simulink model "vRTHS_2024"  (R2025b)
settings: Solver=ode4  StartTime=0.0  StopTime=tend  FixedStep=dt_rths  RelTol=1e-3  EnableMultiTasking=on
values from neighbouring files (symbols this model uses):
  a1_beta0 = 2.1283e+13    (= 21283000000000)    [F1_input_file.m]
  a2 = 4.2297e+06    (= 4229700)    [F1_input_file.m]
  a3 = 3.3        + 1.3   * nom *randn(1,1)    [F1_input_file.m]
  A_ns = [     zeros(n) eye(n) ... (first row only)    [F1_input_file.m]
  AA_R = [zeros(dof)        eye(dof) ... (first row only)    [F1_Modifications.m]
  B_ns = [     zeros(n,1)      zeros(n) ... (first row only)    [F1_input_file.m]
  b_th = 0.13    [RUN_vRTHS_demo_new.m]
  BB_R = [zeros(dof,1) ... (first row only)    [F1_Modifications.m]
  beta1 = 425        + 3.3   * nom *randn(1,1)    [F1_input_file.m]
  beta2 = 9.9976e+04 + 3.3e3 * nom *randn(1,1)    [F1_input_file.m]
  c_e = 2*z_e*m_e*sqrt(KE(1,1)/m_e)    [F1_input_file.m]
  C_ns = [     eye(n)              zeros(n) ... (first row only)    [F1_input_file.m]
  CC_R = [ eye(dof)   zeros(dof) ... (first row only)    [F1_Modifications.m]
  CE = zeros(n)    [F1_input_file.m]
  consider_damage = 0    [RUN_vRTHS_demo_new.m]
  D_ns = [     zeros(n,1)            zeros(n) ... (first row only)    [F1_input_file.m]
  DD_R = [zeros(2*dof,1) ... (first row only)    [F1_Modifications.m]
  dt_rths = 0.000244140625    [Plant.mat]    (also in RUN_vRTHS_demo_new.m)
  E_sw = 1    [F1_input_file.m]
  eq_intensity = .4    (= 0.4)    [F1_input_file.m]
  fs = 4096    [RUN_vRTHS_demo_new.m]
  gain = 1.0261    [F1_input_file.m]
  Gsnsr_DT = 1    [F1_input_file.m]
  Gsnsr_FT = 1    [F1_input_file.m]
  k_e = 1190e3    (= 1190000)    [F1_input_file.m]
  KE = zeros(n)    [F1_input_file.m]
  m_e = m_e*1.3    [F1_Modifications.m]    (also in F1_input_file.m = 29.13)
  ME = ME*1.3    [F1_Modifications.m]    (also in F1_input_file.m = zeros(n))
  modified = 1    [RUN_vRTHS_demo_new.m]
  sat_limit_lower = -3.8    [F1_input_file.m]
  sat_limit_upper = +3.8    (= 3.8)    [F1_input_file.m]
  Seed_snr = rng(seed)    [F1_input_file.m]
  tend = 90    [F1_input_file.m]
undefined symbols (not defined in the file or in its folder): Acd, Apred_mod, Bcd, Bpred_mod, Ccd, Cpred_mod, Dcd, digital_cntrlr, digital_cntrlr2, Dpred_mod
libraries: simulink x3, cstblocks x1, rtwinlib x1
settings Model: SimulationMode=accelerator  Creator=IISL_0175  LastModifiedBy=Victus
settings SolverCC: AlgebraicLoopSolver=TrustRegion
settings DataIOCC: SaveFormat=StructureWithTime  ReturnWorkspaceOutputs=off
settings OptimizationCC: LifeSpan=inf
settings DebuggingCC: InheritedTsInSrcMsg=none  UnconnectedInputMsg=warning  UnconnectedOutputMsg=warning  UnconnectedLineMsg=warning  SFUnexpectedBacktrackingDiag=warning  SFNoUnconditionalDefaultTransitionDiag=warning  SFExecutionAtInitializationDiag=none  ArithmeticOperatorsInVariantConditions=warning
settings HardwareCC: ProdBitPerSizeT=32.0  ProdBitPerPtrDiffT=32.0  ProdWordSize=32.0  ProdHWDeviceType=Specified
settings SFSimCC: SimUseLocalCustomCode=off  CustomCodeUndefinedFunction=UseInterfaceOnly
settings RTWCC: RTWUseLocalCustomCode=off  GPUComputeCapability=3.5
settings CodeAppCC: StateflowObjectComments=on
settings GRTTargetCC: TargetLangStandard=C89/C90 (ANSI)
settings ConfigComp: CovMetricSettings=dw  CovSaveCumulativeToWorkspaceVar=on  CovSaveSingleToWorkspaceVar=on  CovExternalEMLEnable=off

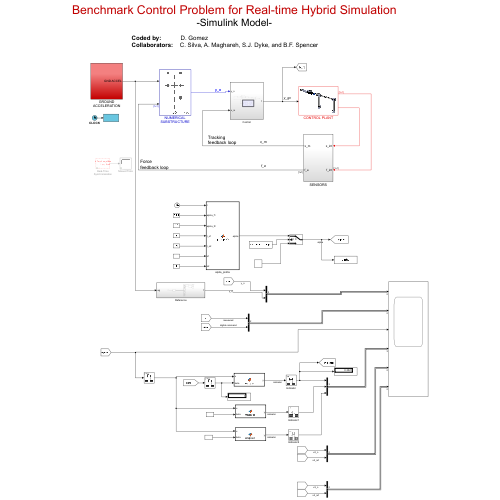
[thumbnail: Simulink's stored preview of the top-level diagram]
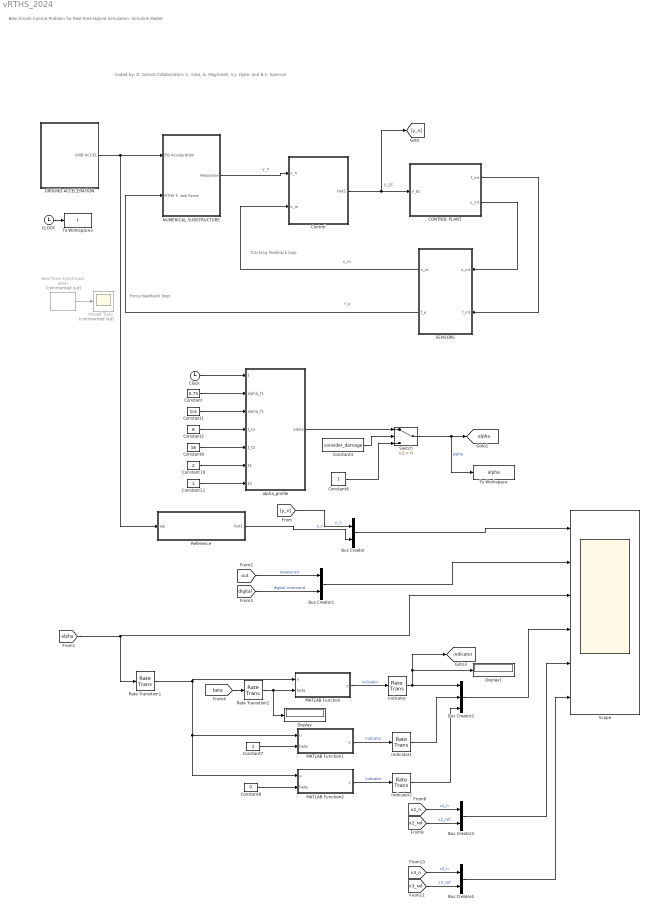
== system vRTHS_2024 ==
  note: Force
      | feedback loop
  note: Benchmark Control Problem for Real-time Hybrid Simulation
      | -Simulink Model-
  note: Coded by: D. Gomez
      | Collaborators: C. Silva, A. Maghareh, S.J. Dyke, and B.F. Spencer
  note: Tracking feedback loop
  note: y_n
  note: y_gc
  note: f_e
  note: x_m
  Bus Creator{,1,3..4} (4 alike) : BusCreator  Inputs=2
  Bus Creator2 : BusCreator  Inputs=3
  CLOCK : Clock
  CONTROL PLANT : Subsystem
      mask Display: image(imread('PlantSW2.PNG'));
  Clock : Clock
  Constant : Constant  Value=0.75
  Constant1 : Constant  Value=0.5
  Constant10 : Constant  Value=2
  Constant11 : Constant
  Constant2 : Constant  Value=8
  Constant3 : Constant  Value=consider_damage
  Constant6 : Constant
  Constant7 : Constant
  Constant8 : Constant  Value=0
  Constant9 : Constant  Value=16
  Control : Subsystem
  Display : Display
  Display1 : Display
  GROUND ACCELERATION : Subsystem
  Indicator : RateTransition
  Indicator1 : RateTransition
  Indicator2 : RateTransition
  MATLAB Function : MATLAB Function  TreatAsAtomicUnit=on  SystemSampleTime=100/fs
  MATLAB Function1 : MATLAB Function  TreatAsAtomicUnit=on  SystemSampleTime=100/fs
  MATLAB Function2 : MATLAB Function  TreatAsAtomicUnit=on  SystemSampleTime=100/fs
  Missed Ticks : Scope  Commented=on
      settings: TimeSpan=10  ActiveDisplayYMinimum=-51.75  ActiveDisplayYMaximum=465.75  DataLoggingSaveFormat=Structure
  NUMERICAL SUBSTRUCTURE : Subsystem
      mask Display: image(imread('Num_sub.png'));
  Rate Transition1 : RateTransition
  Rate Transition2 : RateTransition
  Real-Time Synchronization : rtwinlib/Real-Time Synchronization  Commented=on  SampleTime=dt_rths  MaxMissedTicks=10000  ShowMissedTicks=on  YieldWhenWaiting=off
  Reference : Subsystem
  SENSORS : Subsystem
  Scope : Scope  NumInputPorts=6
      settings: ActiveDisplayString=3  ActiveDisplayYMinimum=0.9  ActiveDisplayYMaximum=1.1  DataLoggingVariableName=ScopeData5
  Switch : Switch  Criteria=u2 > Threshold  SaturateOnIntegerOverflow=off  InputSameDT=off
  To Workspace : ToWorkspace  VariableName=alpha  SaveFormat=Timeseries  SampleTime=-1
  To Workspace3 : ToWorkspace  VariableName=t  SampleTime=-1
  alpha_profile : MATLAB Function  TreatAsAtomicUnit=on
  tag scope: alpha=global, indicator=global
  wires:
  CLOCK/1 -> To Workspace3/1
  CONTROL PLANT/2(x_int) -> SENSORS/1(x_int)
  SENSORS/2("f_e ") -> NUMERICAL SUBSTRUCTURE/2(RTHS feedback Force)
  Control/1(Out1) -> [y_n], CONTROL PLANT/1(y_gc)
  Real-Time Synchronization/1 -> Missed Ticks/1
  GROUND ACCELERATION/1(GND ACCEL) -> Reference/1(ag), NUMERICAL SUBSTRUCTURE/1(EQ Acceleration)
  CONTROL PLANT/1(f_int) -> SENSORS/2(f_int)
  Switch/1 -> To Workspace/1, [alpha]  "alpha"
  Constant/1 -> alpha_profile/2(alpha_f1)
  Clock/1 -> alpha_profile/1(t)
  alpha_profile/1(alpha) -> Switch/1
  Constant11/1 -> alpha_profile/7(k2)
  Constant1/1 -> alpha_profile/3(alpha_f2)
  Constant6/1 -> Switch/3
  Constant2/1 -> alpha_profile/4(t_s1)
  Constant9/1 -> alpha_profile/5(t_s2)
  Constant10/1 -> alpha_profile/6(k1)
  Bus Creator3/1 -> Scope/5
  Bus Creator2/1 -> Scope/4
  MATLAB Function/1(y) -> Indicator/1  "indicator"
  Indicator1/1 -> Bus Creator2/2
  Bus Creator1/1 -> Scope/2
  Bus Creator4/1 -> Scope/6
  Rate Transition1/1 -> MATLAB Function2/1(u), MATLAB Function1/1(u), MATLAB Function/1(u)
  Bus Creator/1 -> Scope/1
  Rate Transition2/1 -> Display/1, MATLAB Function/2(beta)
  Constant7/1 -> MATLAB Function1/2(beta)
  [digital] -> Bus Creator1/2  "digital command"
  [x3_n] -> Bus Creator4/1  "x3_n"
  [x3_ref] -> Bus Creator4/2  "x3_ref"
  [x2_ref] -> Bus Creator3/2  "x2_ref"
  [out] -> Bus Creator1/1  "measured"
  [y_n] -> Bus Creator/1  "y_n"
  Constant8/1 -> MATLAB Function2/2(beta)
  [x2_n] -> Bus Creator3/1  "x2_n"
  [alpha] -> Rate Transition1/1, Scope/3
  MATLAB Function1/1(y) -> Indicator1/1  "indicator"
  Indicator2/1 -> Bus Creator2/3
  Reference/1(Out1) -> Bus Creator/2  "y_r"
  Indicator/1 -> [indicator], Display1/1, Bus Creator2/1
  [beta] -> Rate Transition2/1
  MATLAB Function2/1(y) -> Indicator2/1  "indicator"
  SENSORS/1(x_m) -> Control/2(x_m)
  NUMERICAL SUBSTRUCTURE/1(Response) -> Control/1(y_n)
  Constant3/1 -> Switch/2

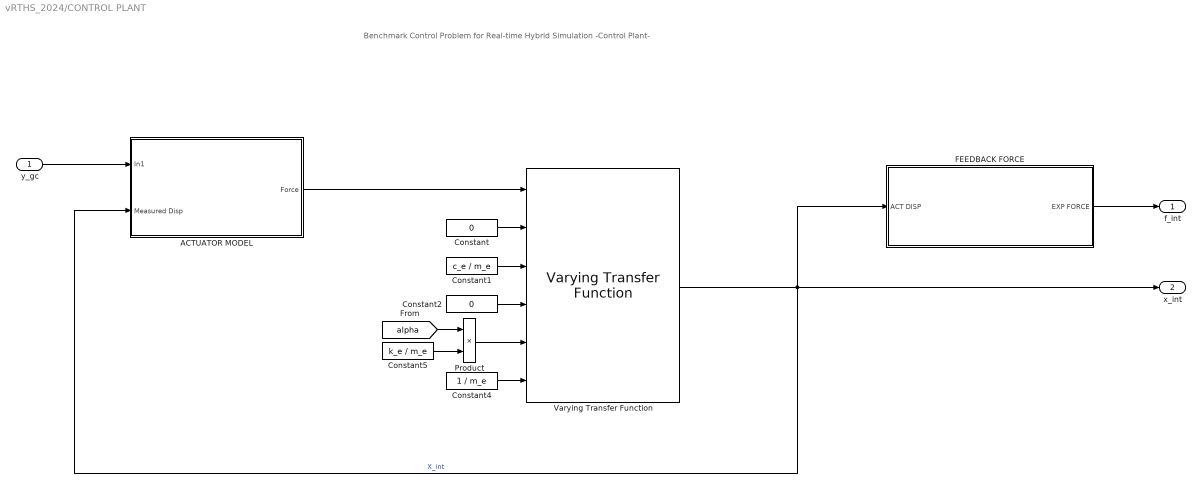
== system vRTHS_2024/CONTROL PLANT ==
  note: Benchmark Control Problem for Real-time Hybrid Simulation
      | -Control Plant-
  y_gc : Inport
  ACTUATOR MODEL : Subsystem
      mask Display: image(imread('ActuatorSW2.PNG'));
  Constant : Constant  Value=0
  Constant1 : Constant  Value=c_e / m_e
  Constant2 : Constant  Value=0
  Constant4 : Constant  Value=1 / m_e
  Constant5 : Constant  Value=k_e / m_e
  FEEDBACK FORCE : Subsystem
  Product : Product
  Varying Transfer Function : cstblocks/Linear Parameter Varying/Varying Transfer Function  N=2  Feedthrough=on
  f_int : Outport
  x_int : Outport  Port=2
  wires:
  y_gc/1 -> ACTUATOR MODEL/1(In1)
  Varying Transfer Function/1 -> FEEDBACK FORCE/1(ACT DISP), x_int/1, ACTUATOR MODEL/2(Measured Disp)  "X_int"
  ACTUATOR MODEL/1(Force) -> Varying Transfer Function/1
  FEEDBACK FORCE/1(EXP FORCE) -> f_int/1
  Constant4/1 -> Varying Transfer Function/6
  [alpha] -> Product/1
  Product/1 -> Varying Transfer Function/5
  Constant1/1 -> Varying Transfer Function/3
  Constant5/1 -> Product/2
  Constant/1 -> Varying Transfer Function/2
  Constant2/1 -> Varying Transfer Function/4

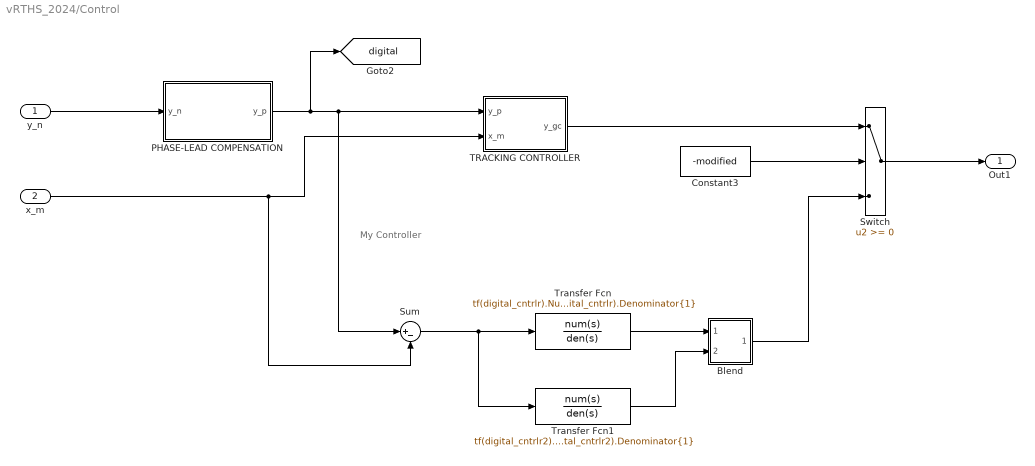
== system vRTHS_2024/Control ==
  note: My Controller
  y_n : Inport
  x_m : Inport  Port=2
  Blend : Subsystem
  Constant3 : Constant  Value=-modified
  PHASE-LEAD COMPENSATION : Subsystem
  Sum : Sum  Inputs=|+-
  Switch : Switch  SaturateOnIntegerOverflow=off  InputSameDT=off
  TRACKING CONTROLLER : Subsystem
  Transfer Fcn : TransferFcn  Numerator=tf(digital_cntrlr).Numerator{1}  Denominator=tf(digital_cntrlr).Denominator{1}
  Transfer Fcn1 : TransferFcn  Numerator=tf(digital_cntrlr2).Numerator{1}  Denominator=tf(digital_cntrlr2).Denominator{1}
  Out1 : Outport
  tag scope: digital=global
  wires:
  x_m/1 -> Sum/2, TRACKING CONTROLLER/2(x_m)
  Sum/1 -> Transfer Fcn1/1, Transfer Fcn/1
  Transfer Fcn1/1 -> Blend/2(In2)
  Transfer Fcn/1 -> Blend/1(In1)
  TRACKING CONTROLLER/1(y_gc) -> Switch/1
  Blend/1(Out1) -> Switch/3
  PHASE-LEAD COMPENSATION/1(y_p) -> [digital], Sum/1, TRACKING CONTROLLER/1(y_p)
  Constant3/1 -> Switch/2
  Switch/1 -> Out1/1
  y_n/1 -> PHASE-LEAD COMPENSATION/1(y_n)

== system vRTHS_2024/GROUND ACCELERATION ==
  note: Benchmark Control Problem for Real-time Hybrid Simulation
      | -Ground Acceleration-
  GROUND ACCELERATION : ToWorkspace  VariableName=EQ_input  SampleTime=-1
  INPUT SELECTOR : MultiPortSwitch  Inputs=4  SaturateOnIntegerOverflow=off  InputSameDT=off
  "RECORD " : Subsystem
  SCALING : Gain  Gain=eq_intensity  Multiplication=Matrix(K*u)
  SWITCH CONSTANT : Constant  Value=E_sw
  GND ACCEL : Outport
  wires:
  INPUT SELECTOR/1 -> SCALING/1
  SWITCH CONSTANT/1 -> INPUT SELECTOR/1
  "RECORD "/1(El Centro) -> INPUT SELECTOR/2
  "RECORD "/2(Kobe) -> INPUT SELECTOR/3
  "RECORD "/3(Morgan) -> INPUT SELECTOR/4
  SCALING/1 -> GROUND ACCELERATION/1, GND ACCEL/1
  "RECORD "/4(Chirp) -> INPUT SELECTOR/5

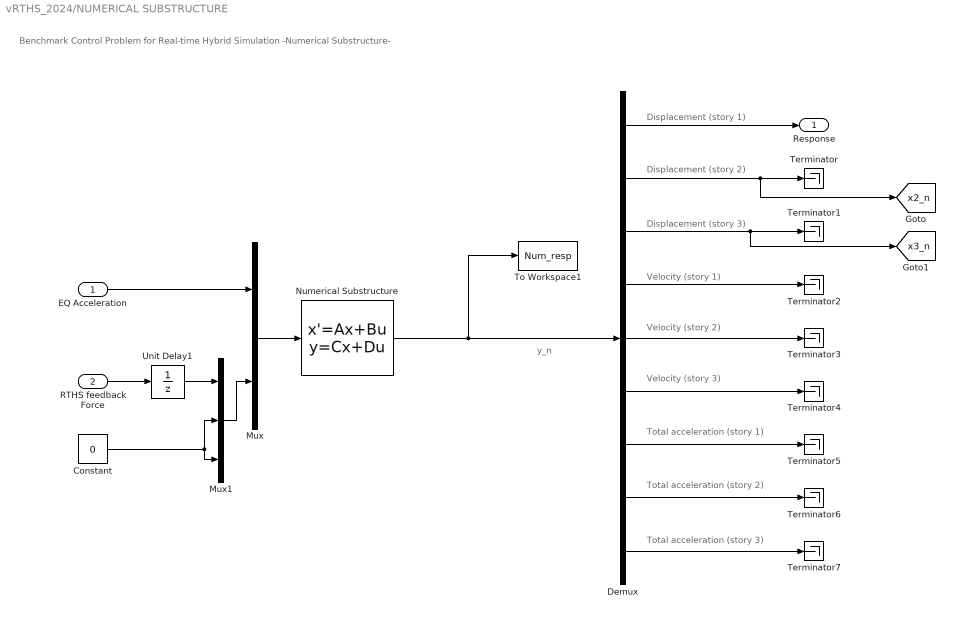
== system vRTHS_2024/NUMERICAL SUBSTRUCTURE ==
  note: y_n
  note: Benchmark Control Problem for Real-time Hybrid Simulation
      | -Numerical Substructure-
  note: Velocity (story 3)
  note: Displacement (story 3)
  note: Displacement (story 1)
  note: Total acceleration (story 1)
  note: Velocity (story 1)
  note: Velocity (story 2)
  note: Total acceleration (story 3)
  note: Displacement (story 2)
  note: Total acceleration (story 2)
  EQ Acceleration : Inport
  RTHS feedback Force : Inport  Port=2
  Constant : Constant  Value=0
  Demux : Demux  Outputs=9
  Mux : Mux  Inputs=2
  Mux1 : Mux  Inputs=3
  Numerical Substructure : StateSpace  A=A_ns  B=B_ns  C=C_ns  D=D_ns  InitialCondition=0
  Terminator{,1..7} (8 alike) : Terminator
  To Workspace1 : ToWorkspace  VariableName=Num_resp  SaveFormat=Timeseries  SampleTime=-1
  Unit Delay1 : UnitDelay  SampleTime=-1  HasFrameUpgradeWarning=on
  Response : Outport
  tag scope: x2_n=global, x3_n=global
  wires:
  Mux/1 -> Numerical Substructure/1
  EQ Acceleration/1 -> Mux/1
  RTHS feedback Force/1 -> Unit Delay1/1
  Numerical Substructure/1 -> To Workspace1/1, Demux/1
  Demux/2 -> [x2_n], Terminator/1
  Demux/7 -> Terminator5/1
  Demux/8 -> Terminator6/1
  Demux/9 -> Terminator7/1
  Demux/4 -> Terminator2/1
  Demux/6 -> Terminator4/1
  Demux/5 -> Terminator3/1
  Demux/1 -> Response/1
  Demux/3 -> [x3_n], Terminator1/1
  Constant/1 -> Mux1/2, Mux1/3
  Mux1/1 -> Mux/2
  Unit Delay1/1 -> Mux1/1

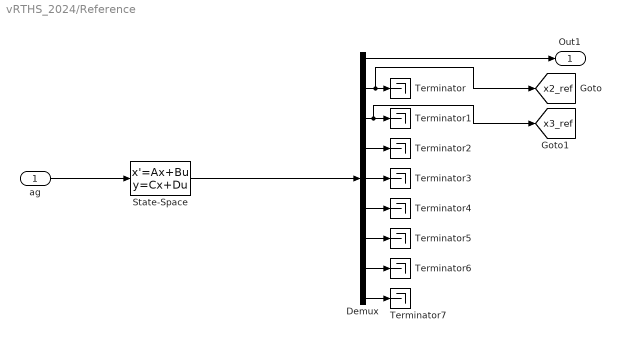
== system vRTHS_2024/Reference ==
  ag : Inport
  Demux : Demux  Outputs=9
  State-Space : StateSpace  A=AA_R  B=BB_R  C=CC_R  D=DD_R  InitialCondition=0
  Terminator{,1..7} (8 alike) : Terminator
  Out1 : Outport
  tag scope: x2_ref=global, x3_ref=global
  wires:
  Demux/7 -> Terminator5/1
  Demux/6 -> Terminator4/1
  Demux/8 -> Terminator6/1
  Demux/9 -> Terminator7/1
  Demux/3 -> [x3_ref], Terminator1/1
  Demux/4 -> Terminator2/1
  Demux/2 -> [x2_ref], Terminator/1
  Demux/5 -> Terminator3/1
  State-Space/1 -> Demux/1
  ag/1 -> State-Space/1
  Demux/1 -> Out1/1

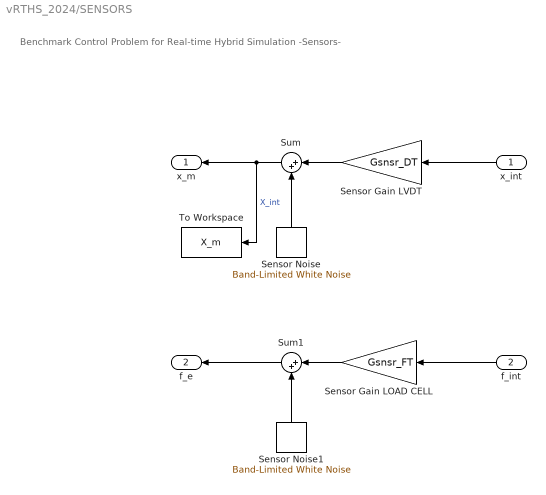
== system vRTHS_2024/SENSORS ==
  note: Benchmark Control Problem for Real-time Hybrid Simulation
      | -Sensors-
  x_int : Inport
  f_int : Inport  Port=2
  Sensor Noise : simulink/Sources/Band-Limited White Noise  Cov=rms_noise_DT  Ts=dt_rths  seed=double(Seed_snr.Seed)
  Sensor Noise1 : simulink/Sources/Band-Limited White Noise  Cov=rms_noise_FT  Ts=dt_rths  seed=double(Seed_snr.Seed)
  Sensor Gain LVDT : Gain  Gain=Gsnsr_DT  SaturateOnIntegerOverflow=on  OutDataTypeStr=Inherit: Same as input  ParamDataTypeStr=Inherit: Same as input
  Sensor Gain LOAD CELL : Gain  Gain=Gsnsr_FT  SaturateOnIntegerOverflow=on  OutDataTypeStr=Inherit: Same as input  ParamDataTypeStr=Inherit: Same as input
  Sum : Sum  Inputs=|++  InputSameDT=on  SaturateOnIntegerOverflow=on  OutDataTypeStr=Inherit: Same as first input
  Sum1 : Sum  Inputs=|++  InputSameDT=on  SaturateOnIntegerOverflow=on  OutDataTypeStr=Inherit: Same as first input
  To Workspace : ToWorkspace  VariableName=X_m  SaveFormat=Timeseries  SampleTime=-1
  x_m : Outport
  "f_e " : Outport  Port=2
  wires:
  Sensor Gain LVDT/1 -> Sum/1
  Sensor Noise/1 -> Sum/2
  x_int/1 -> Sensor Gain LVDT/1
  Sensor Gain LOAD CELL/1 -> Sum1/1
  Sum1/1 -> "f_e "/1
  Sensor Noise1/1 -> Sum1/2
  f_int/1 -> Sensor Gain LOAD CELL/1
  Sum/1 -> x_m/1, To Workspace/1  "X_int"

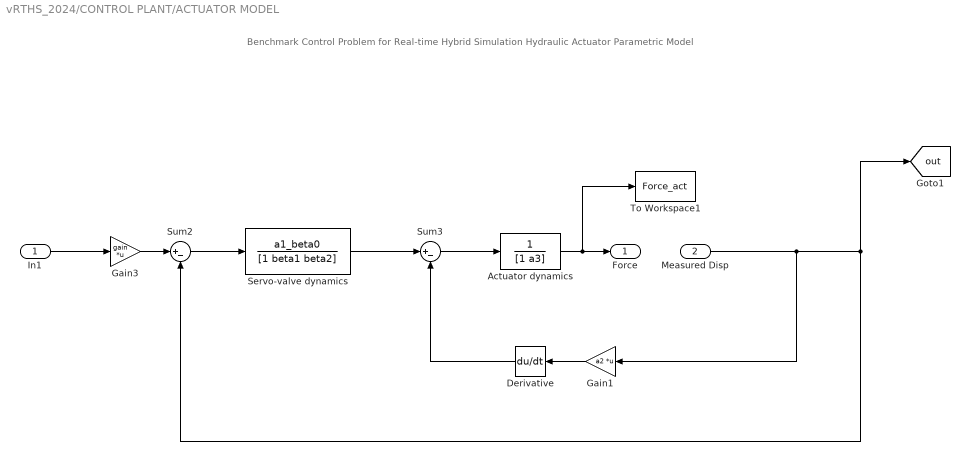
== system vRTHS_2024/CONTROL PLANT/ACTUATOR MODEL ==
  note: Benchmark Control Problem for Real-time Hybrid Simulation
      | Hydraulic Actuator Parametric Model
  In1 : Inport
  Measured Disp : Inport  Port=2
  Actuator dynamics : TransferFcn  Numerator=1  Denominator=[1 a3]
  Derivative : Derivative
  Gain1 : Gain  Gain=a2  Multiplication=Matrix(K*u)
  Gain3 : Gain  Gain=gain  Multiplication=Matrix(K*u)
  Servo-valve dynamics : TransferFcn  Numerator=a1_beta0  Denominator=[1 beta1 beta2]
  Sum2 : Sum  Inputs=|+-
  Sum3 : Sum  Inputs=|+-
  To Workspace1 : ToWorkspace  VariableName=Force_act  SaveFormat=Timeseries  SampleTime=-1
  Force : Outport
  tag scope: out=global
  wires:
  Gain3/1 -> Sum2/1
  Actuator dynamics/1 -> To Workspace1/1, Force/1
  Servo-valve dynamics/1 -> Sum3/1
  In1/1 -> Gain3/1
  Sum2/1 -> Servo-valve dynamics/1
  Gain1/1 -> Derivative/1
  Derivative/1 -> Sum3/2
  Sum3/1 -> Actuator dynamics/1
  Measured Disp/1 -> [out], Sum2/2, Gain1/1

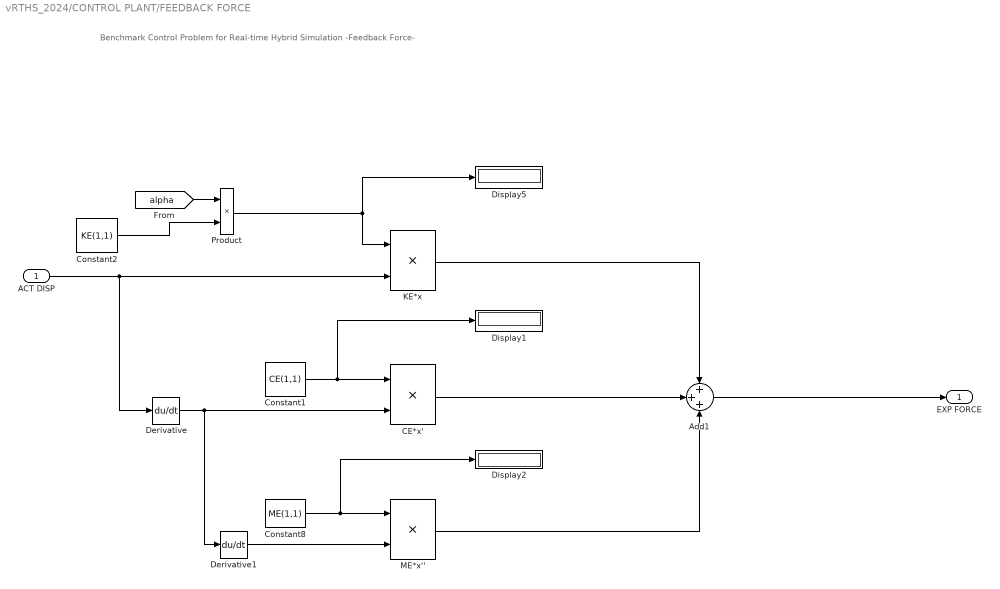
== system vRTHS_2024/CONTROL PLANT/FEEDBACK FORCE ==
  note: Benchmark Control Problem for Real-time Hybrid Simulation
      | -Feedback Force-
  ACT DISP : Inport
  Add1 : Sum  Inputs=+++
  CE*x' : Product  RndMeth=Zero
  Constant1 : Constant  Value=CE(1,1)  VectorParams1D=off
  Constant2 : Constant  Value=KE(1,1)  VectorParams1D=off
  Constant8 : Constant  Value=ME(1,1)  VectorParams1D=off
  Derivative : Derivative
  Derivative1 : Derivative
  Display1 : Display
  Display2 : Display
  Display5 : Display
  KE*x : Product  RndMeth=Zero
  ME*x'' : Product  RndMeth=Zero
  Product : Product
  EXP FORCE : Outport
  wires:
  Constant1/1 -> Display1/1, CE*x'/1
  Constant8/1 -> Display2/1, ME*x''/1
  ACT DISP/1 -> KE*x/2, Derivative/1
  Derivative/1 -> CE*x'/2, Derivative1/1
  Derivative1/1 -> ME*x''/2
  Add1/1 -> EXP FORCE/1
  KE*x/1 -> Add1/1
  CE*x'/1 -> Add1/2
  ME*x''/1 -> Add1/3
  Product/1 -> Display5/1, KE*x/1
  [alpha] -> Product/1
  Constant2/1 -> Product/2

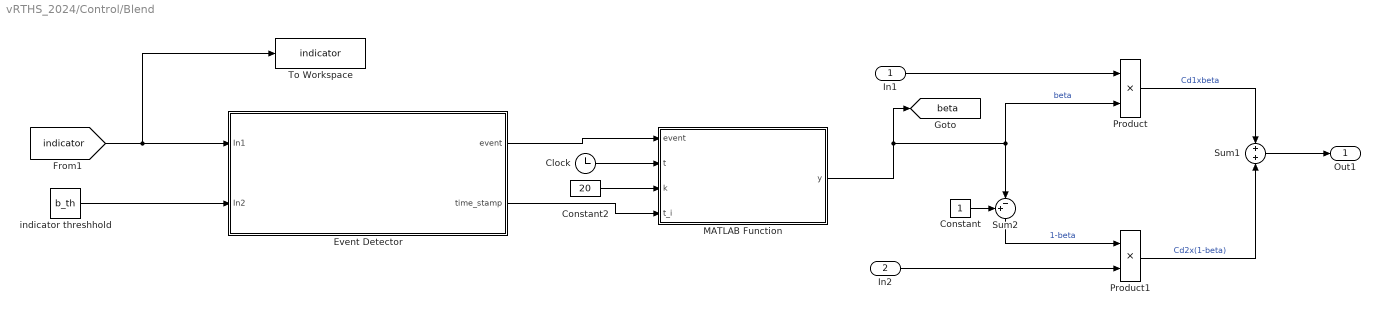
== system vRTHS_2024/Control/Blend ==
  In1 : Inport
  In2 : Inport  Port=2
  Clock : Clock
  Constant : Constant
  Constant2 : Constant  Value=20
  Event Detector : Subsystem
  MATLAB Function : MATLAB Function  TreatAsAtomicUnit=on
  Product : Product
  Product1 : Product
  Sum1 : Sum
  Sum2 : Sum  Inputs=+-|
  To Workspace : ToWorkspace  VariableName=indicator  SaveFormat=Timeseries  SampleTime=-1
  indicator threshhold : Constant  Value=b_th
  Out1 : Outport
  tag scope: beta=global
  wires:
  Sum2/1 -> Product1/1  "1-beta"
  Sum1/1 -> Out1/1
  Product1/1 -> Sum1/2  "Cd2x(1-beta)"
  MATLAB Function/1(y) -> Product/2, Sum2/2, [beta]  "beta"
  Product/1 -> Sum1/1  "Cd1xbeta"
  Constant/1 -> Sum2/1
  In2/1 -> Product1/2
  In1/1 -> Product/1
  Event Detector/2(time_stamp) -> MATLAB Function/4(t_i)
  Constant2/1 -> MATLAB Function/3(k)
  [indicator] -> To Workspace/1, Event Detector/1(In1)
  indicator threshhold/1 -> Event Detector/2(In2)
  Event Detector/1(event) -> MATLAB Function/1(event)
  Clock/1 -> MATLAB Function/2(t)

== system vRTHS_2024/Control/PHASE-LEAD COMPENSATION ==
  note: Benchmark Control Problem for Real-time Hybrid Simulation
      | -Phase-Lead Compensation-
  y_n : Inport
  A/D Converter : Subsystem
  D/A Converter : Subsystem
  Discrete Controller : DiscreteStateSpace  A=Apred_mod  B=Bpred_mod  C=Cpred_mod  D=Dpred_mod  SampleTime=dt_rths
  y_p : Outport
  wires:
  Discrete Controller/1 -> D/A Converter/1(u(k))
  y_n/1 -> A/D Converter/1(y(t))
  A/D Converter/1(y(k)) -> Discrete Controller/1
  D/A Converter/1(u(t)) -> y_p/1

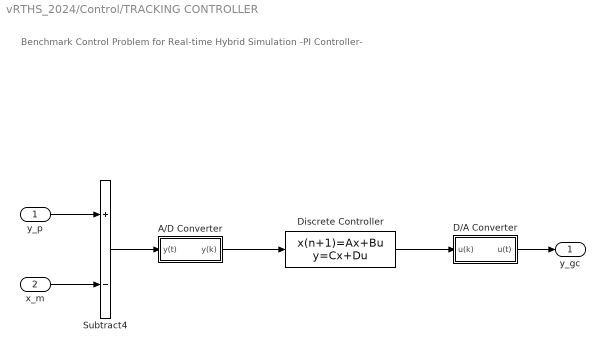
== system vRTHS_2024/Control/TRACKING CONTROLLER ==
  note: Benchmark Control Problem for Real-time Hybrid Simulation
      | -PI Controller-
  y_p : Inport
  x_m : Inport  Port=2
  A/D Converter : Subsystem
  D/A Converter : Subsystem
  Discrete Controller : DiscreteStateSpace  A=Acd  B=Bcd  C=Ccd  D=Dcd  SampleTime=dt_rths
  Subtract4 : Sum  Inputs=+-
  y_gc : Outport
  wires:
  y_p/1 -> Subtract4/1
  Discrete Controller/1 -> D/A Converter/1(u(k))
  Subtract4/1 -> A/D Converter/1(y(t))
  x_m/1 -> Subtract4/2
  A/D Converter/1(y(k)) -> Discrete Controller/1
  D/A Converter/1(u(t)) -> y_gc/1

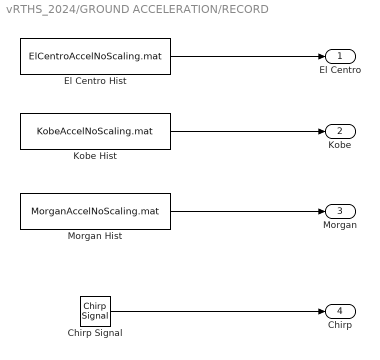
== system vRTHS_2024/GROUND ACCELERATION/RECORD  ==
  Chirp Signal : simulink/Sources/Chirp Signal  f1=f_ini  T=tend  f2=f_end
  El Centro Hist : FromFile  FileName=ElCentroAccelNoScaling.mat
  Kobe Hist : FromFile  FileName=KobeAccelNoScaling.mat
  Morgan Hist : FromFile  FileName=MorganAccelNoScaling.mat
  El Centro : Outport
  Kobe : Outport  Port=2
  Morgan : Outport  Port=3
  Chirp : Outport  Port=4
  wires:
  Morgan Hist/1 -> Morgan/1
  Kobe Hist/1 -> Kobe/1
  El Centro Hist/1 -> El Centro/1
  Chirp Signal/1 -> Chirp/1

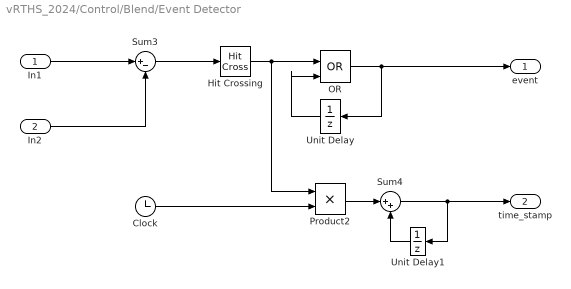
== system vRTHS_2024/Control/Blend/Event Detector ==
  In1 : Inport
  In2 : Inport  Port=2
  Clock : Clock
  Hit Crossing : HitCross  HitCrossingDirection=falling
  OR : Logic  Operator=OR  IconShape=distinctive  AllPortsSameDT=off  OutDataTypeStr=boolean
  Product2 : Product
  Sum3 : Sum  Inputs=|+-
  Sum4 : Sum  Inputs=|++
  Unit Delay : UnitDelay  SampleTime=-1  HasFrameUpgradeWarning=on
  Unit Delay1 : UnitDelay  SampleTime=-1  HasFrameUpgradeWarning=on
  event : Outport
  time_stamp : Outport  Port=2
  wires:
  OR/1 -> event/1, Unit Delay/1
  Sum3/1 -> Hit Crossing/1
  Unit Delay/1 -> OR/2
  Sum4/1 -> time_stamp/1, Unit Delay1/1
  Unit Delay1/1 -> Sum4/2
  Hit Crossing/1 -> Product2/1, OR/1
  Clock/1 -> Product2/2
  Product2/1 -> Sum4/1
  In2/1 -> Sum3/2
  In1/1 -> Sum3/1

== system vRTHS_2024/Control/PHASE-LEAD COMPENSATION/A//D Converter ==
  y(t) : Inport
  Quantizer : Quantizer  QuantizationInterval=quantize_int
  Saturation : Saturate  UpperLimit=sat_limit_upper  LowerLimit=sat_limit_lower
  y(k) : Outport
  wires:
  Saturation/1 -> Quantizer/1
  Quantizer/1 -> y(k)/1
  y(t)/1 -> Saturation/1

== system vRTHS_2024/Control/PHASE-LEAD COMPENSATION/D//A Converter ==
  u(k) : Inport
  Quantizer : Quantizer  QuantizationInterval=quantize_int
  Saturation : Saturate  UpperLimit=sat_limit_upper  LowerLimit=sat_limit_lower
  u(t) : Outport
  wires:
  Saturation/1 -> u(t)/1
  Quantizer/1 -> Saturation/1
  u(k)/1 -> Quantizer/1

== system vRTHS_2024/Control/TRACKING CONTROLLER/A//D Converter ==
  y(t) : Inport
  Quantizer : Quantizer  QuantizationInterval=quantize_int
  Saturation : Saturate  UpperLimit=sat_limit_upper  LowerLimit=sat_limit_lower
  y(k) : Outport
  wires:
  Saturation/1 -> Quantizer/1
  Quantizer/1 -> y(k)/1
  y(t)/1 -> Saturation/1

== system vRTHS_2024/Control/TRACKING CONTROLLER/D//A Converter ==
  u(k) : Inport
  Quantizer : Quantizer  QuantizationInterval=quantize_int
  Saturation : Saturate  UpperLimit=sat_limit_upper  LowerLimit=sat_limit_lower
  u(t) : Outport
  wires:
  Saturation/1 -> u(t)/1
  Quantizer/1 -> Saturation/1
  u(k)/1 -> Quantizer/1

== matlab function vRTHS_2024/MATLAB Function ==
  data: u input; y output; beta input
function y = wrapper(u, beta)
%#codegen
coder.extrinsic('sim_helper');  % run helper in MATLAB during simulation
y = 0;                        % preinit to fix type/size
y = sim_helper(u, beta);

== matlab function vRTHS_2024/alpha_profile ==
  data: t input; alpha output; alpha_f1 input; alpha_f2 input; t_s1 input; t_s2 input; k1 input; k2 input
function alpha = alpha_profile(t, alpha_f1, alpha_f2, t_s1, t_s2, k1, k2)

    tt = max(t,0);
    term1 = (1 - alpha_f1) ./ (1 + exp(-k1 .* (tt - t_s1)));
    term2 = (alpha_f1 - alpha_f2) ./ (1 + exp(-k2 .* (tt - t_s2)));
    
    alpha = 1 - term1 - term2;

end

== matlab function vRTHS_2024/MATLAB Function1 ==
  data: u input; y output; beta input
function y = wrapper(u, beta)
%#codegen
coder.extrinsic('sim_helper');  % run helper in MATLAB during simulation
y = 0;                        % preinit to fix type/size
y = sim_helper(u, beta);

== matlab function vRTHS_2024/MATLAB Function2 ==
  data: u input; y output; beta input
function y = wrapper(u, beta)
%#codegen
coder.extrinsic('sim_helper');  % run helper in MATLAB during simulation
y = 0;                        % preinit to fix type/size
y = sim_helper(u, beta);

== matlab function vRTHS_2024/Control/Blend/MATLAB Function ==
  data: event input; t input; y output; k input; t_i input
function y = beta_value(event, t, k, t_i)
%#codegen
% event : logical/boolean (1 -> force output to 0)
% t     : current sim time from a Clock block (scalar)
% k     : steepness
% t_s   : center time of the S-curve

    % Ensure scalar time (Clock already gives a scalar)
    tt = t;

    if ~event
        % If the event is active, force output to zero and exit.
        y = 1;
        return;
    end
    t_s = t_i + 5/k;  % pushes the steepest point to insure smooth transition (2.5/k is an emperical value)
    % Otherwise, logistic S-shaped value
    y = 1 - 1 / (1 + exp(-k * (tt - t_s)));
end
